simulink model "SRA_P2_derivativo_rampa"  (R2026b)
settings: Solver=VariableStepAuto
libraries: simulink x1
settings Model: Creator=paull  LastModifiedBy=enriq

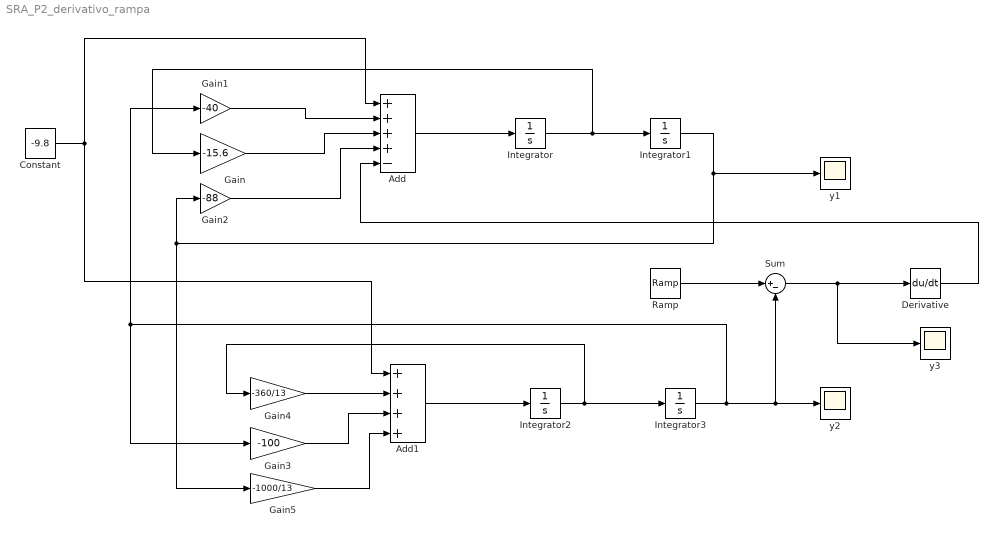
== system SRA_P2_derivativo_rampa ==
  Add : Sum  Inputs=++++-
  Add1 : Sum  Inputs=++++
  Constant : Constant  Value=-9.8
  Derivative : Derivative  CoefficientInTFapproximation=5
  Gain : Gain  Gain=-15.6
  Gain1 : Gain  Gain=-40
  Gain2 : Gain  Gain=-88
  Gain3 : Gain  Gain=-100
  Gain4 : Gain  Gain=-360/13
  Gain5 : Gain  Gain=-1000/13
  Integrator{,1..3} (4 alike) : Integrator
  Ramp : simulink/Sources/Ramp  slope=2  start=0  InitialOutput=0
  Sum : Sum  Inputs=|+-
  y1 : Scope
      settings: ActiveDisplayYMinimum=-141.40465215898942  ActiveDisplayYMaximum=293.11158093061181
  y2 : Scope
      settings: ActiveDisplayYMinimum=-0.12452593572736521  ActiveDisplayYMaximum=0.14871704617306764
  y3 : Scope
      settings: ActiveDisplayYMinimum=-3.4598078789728861  ActiveDisplayYMaximum=12.39879247857376  DataLoggingVariableName=ScopeData2
  wires:
  Integrator1/1 -> Gain5/1, Gain2/1, y1/1
  Integrator/1 -> Integrator1/1, Gain/1
  Add/1 -> Integrator/1
  Gain2/1 -> Add/4
  Gain/1 -> Add/3
  Integrator3/1 -> Gain3/1, Gain1/1, Sum/2, y2/1
  Integrator2/1 -> Gain4/1, Integrator3/1
  Constant/1 -> Add/1, Add1/1
  Gain1/1 -> Add/2
  Add1/1 -> Integrator2/1
  Gain4/1 -> Add1/2
  Gain3/1 -> Add1/3
  Gain5/1 -> Add1/4
  Sum/1 -> Derivative/1, y3/1
  Ramp/1 -> Sum/1
  Derivative/1 -> Add/5
